simulink model "effect_of_source_inductance_in_rl_load"  (R2024a)
settings: Solver=VariableStepAuto  StartTime=0.0  StopTime=0.06  RelTol=1e-3
undefined symbols (not defined in the file): a
libraries: spsVoltageMeasurementLib x5, spsThyristorLib x4, spsCurrentMeasurementLib x3, spsSeriesRLCBranchLib x3, spsACVoltageSourceLib x1, sps_lib x1
settings Model: Creator=Adithyan  LastModifiedBy=Adithyan

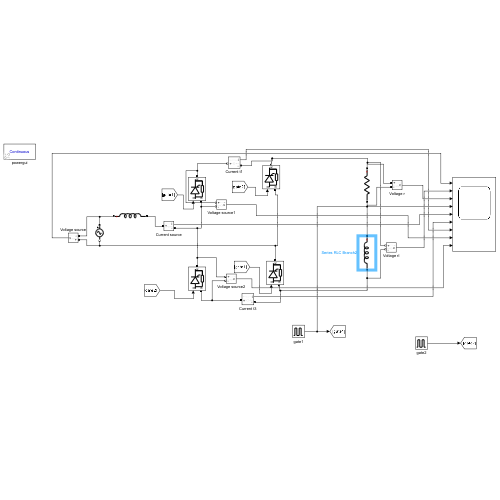
[thumbnail: Simulink's stored preview of the top-level diagram]
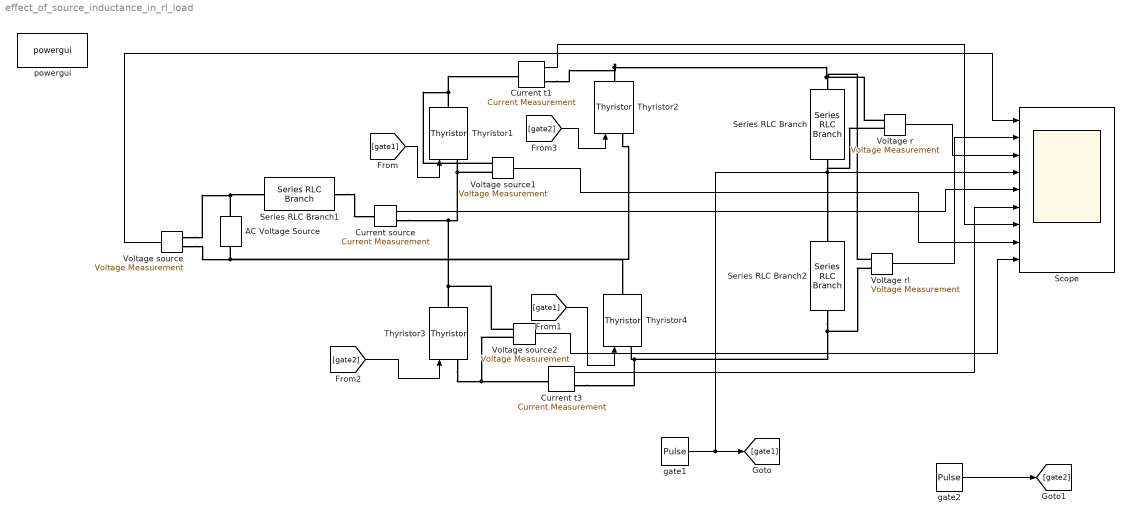
== system effect_of_source_inductance_in_rl_load ==
  AC Voltage Source : spsACVoltageSourceLib/AC Voltage Source  Amplitude=24  Phase=0  Frequency=50  SampleTime=0  Measurements=None  BusType=swing  Pref=10e3  Qref=0  Qmin=-inf  Qmax=+inf
  Current source : spsCurrentMeasurementLib/Current Measurement  PhasorSimulation=off  OutputType=Complex  PSBequivalent=0
  Current t1 : spsCurrentMeasurementLib/Current Measurement  PhasorSimulation=off  OutputType=Complex  PSBequivalent=0
  Current t3 : spsCurrentMeasurementLib/Current Measurement  PhasorSimulation=off  OutputType=Complex  PSBequivalent=0
  Scope : Scope  NumInputPorts=9
  Series RLC Branch : spsSeriesRLCBranchLib/Series RLC Branch  LConnTagsString=__new0  RConnTagsString=__new0  BranchType=R  Resistance=100  Inductance=50e-3  SetiL0=off  InitialCurrent=0  Capacitance=1e-6  Setx0=off  InitialVoltage=0  Measurements=Branch voltage and current
  Series RLC Branch1 : spsSeriesRLCBranchLib/Series RLC Branch  LConnTagsString=__new0  RConnTagsString=__new0  BranchType=L  Resistance=1  Inductance=1e-3  SetiL0=off  InitialCurrent=0  Capacitance=1e-6  Setx0=off  InitialVoltage=0  Measurements=None
  Series RLC Branch2 : spsSeriesRLCBranchLib/Series RLC Branch  LConnTagsString=__new0  RConnTagsString=__new0  BranchType=L  Resistance=1  Inductance=10e-3  SetiL0=off  InitialCurrent=0  Capacitance=1e-6  Setx0=off  InitialVoltage=0  Measurements=None
  Thyristor{1..4} (4 alike) : spsThyristorLib/Thyristor  Ron=0.001  Lon=0  Vf=0.8  IC=0  Rs=500  Cs=250e-9  Measurements=off
  Voltage r : spsVoltageMeasurementLib/Voltage Measurement  PhasorSimulation=off  OutputType=Complex  PSBequivalent=0
  Voltage rl : spsVoltageMeasurementLib/Voltage Measurement  PhasorSimulation=off  OutputType=Complex  PSBequivalent=0
  Voltage source : spsVoltageMeasurementLib/Voltage Measurement  PhasorSimulation=off  OutputType=Complex  PSBequivalent=0
  Voltage source1 : spsVoltageMeasurementLib/Voltage Measurement  PhasorSimulation=off  OutputType=Complex  PSBequivalent=0
  Voltage source2 : spsVoltageMeasurementLib/Voltage Measurement  PhasorSimulation=off  OutputType=Complex  PSBequivalent=0
  gate1 : DiscretePulseGenerator  PulseType=Time based  Period=1/50  PulseWidth=5  PhaseDelay=(a/360)*1/50
  gate2 : DiscretePulseGenerator  PulseType=Time based  Period=1/50  PulseWidth=5  PhaseDelay=((a/360)*1/50)+1/100
  powergui : sps_lib/powergui  Priority=1  SimulationMode=Continuous  SampleTime=50e-6  frequency=60  Iterations=50  frequencyindice=50  Pbase=100e6  ErrMax=1e-4  UnitsV=kV  UnitsW=MW  buscounter=0  FunctionMessages=off  echomessages=off  EnableUseOfTLC=off  CurrentSourceSwitches=off  DisableSnubberDevices=off  DisableRonSwitches=off  DisableVfSwitches=off  DisplayEquations=off  AutomaticDiscreteSolvers=off  SolverType=Tustin/Backward Euler (TBE)  Interpol=off  ExternalGateDelay=off  methode=off  Ts=100  x0status=blocks  SPID=on  SwTol=0  HookPort=off  NonlinearTolerance=1e-4  nMaxIteration=100  ContinueOnMaxIteration=off  RestoreLinks=warning  ResistiveCurrentMeasurement=off  Frange=[0:2:500]  Ylog=off  Xlog=on  ShowGrid=off  save=off  variable=ZData  structure=0  ZoomFFT=off  StartTime=0.0  cycles=1  DisplayStyle=1  fundamental=60  FreqAxis=off  MaxFrequency=1000  frequencyindicesteady=1  RmsSteady=1  display=off
  wires:
  [gate2] -> Thyristor2/1
  Voltage source/1 -> Scope/1
  Voltage r/1 -> Scope/3
  [gate1] -> Thyristor1/1
  [gate1] -> Thyristor4/1
  gate1/1 -> Scope/4, [gate1]
  [gate2] -> Thyristor3/1
  gate2/1 -> [gate2]
  Current t3/1 -> Scope/6
  Voltage rl/1 -> Scope/2
  Current t1/1 -> Scope/7
  Current source/1 -> Scope/5
  Voltage source1/1 -> Scope/8
  Voltage source2/1 -> Scope/9
  connections:
  AC Voltage Source/LConn1 -- Thyristor4/RConn1 -- Thyristor2/LConn1 -- Voltage source/LConn1
  Series RLC Branch2/RConn1 -- Current t3/RConn1 -- Thyristor4/LConn1 -- Voltage rl/LConn2
  Thyristor2/RConn1 -- Voltage rl/LConn1 -- Series RLC Branch/LConn1 -- Voltage r/LConn1 -- Current t1/RConn1
  Thyristor3/RConn1 -- Voltage source2/LConn1 -- Voltage source1/LConn2 -- Thyristor1/LConn1 -- Current source/RConn1
  AC Voltage Source/RConn1 -- Voltage source/LConn2 -- Series RLC Branch1/LConn1
  Series RLC Branch/RConn1 -- Series RLC Branch2/LConn1 -- Voltage r/LConn2
  Series RLC Branch1/RConn1 -- Current source/LConn1
  Thyristor3/LConn1 -- Voltage source2/LConn2 -- Current t3/LConn1
  Thyristor1/RConn1 -- Voltage source1/LConn1 -- Current t1/LConn1
